simulink model "mb_kol_model"  (R2026b)
settings: Solver=ode4  StopTime=T  FixedStep=dt
values from neighbouring files (symbols this model uses):
  M = mb_param(S)    [dogrula_mb.m]    (also in mb_animasyon.m = mb_param(S);  S.mgl = 0; mb_kareler.m; olcum_oku.m = squeeze(m.Data);  if size(M,2) ~= 6, M = M'; end)
  m = [thm; olc(x(1), S.qM); v; u]    [blok_ayrik.m]    (also in dogrula_b2.m = min(numel(t_s), numel(o.t)); dogrula_b2_dt.m = min(numel(t_s), numel(o.t)); dogrula_elk.m = min(numel(t_s), numel(o.t)); mb_animasyon.m = mean(th(son)))
  S = sim_param(q, D(k).ac, kp)    [deney_4a.m]    (also in dogrula_2.m = sim_param(q, h.ac, ref.kp); dogrula_3.m = sim_param(q, h.ac, kp); dogrula_b2.m = sim_param(q, ac, kp); dogrula_b2_dt.m = sim_param(q, ac, kp))
  s = any(C >= 3 & A > 0.5, 3)    [analiz_5b.m]    (also in blok_ayrik.m = sin(2*pi*S.dny_f0*tau); deney_4a.m = fr > 0.5 & fr < 0.5/dt; km_kestir.m = find(t >= tbas, 1); olcum_4b.m = K.t > 0.1)
  Ts = t(2) - t(1)    [km_kestir.m]    (also in tani_Fs.m; tani_JM.m; tani_JM_kol.m; tani_Ks.m)
  X = squeeze(xs.Data);  if size(X,2) ~= 4, X = X'; end    [deney_4a.m]    (also in dogrula_2.m = squeeze(xs.Data); dogrula_3.m = squeeze(xs.Data); dogrula_5a.m = squeeze(xs.Data); dogrula_b2.m)
  Y = abs(fft(y .* (0.5 - 0.5*cos(2*pi*(0:n-1)'/(n-1)))))    [deney_4a.m]    (also in mb_kareler.m = reshape(P(2,:), size(x)) + c(2))
  Z = reshape(P(3,:), size(x)) + c(3)    [mb_kareler.m]
libraries: sm_lib x15, fl_lib x8, nesl_utility x7
settings Model: Creator=safak  LastModifiedBy=safak
settings DataIOCC: Decimation=dec  SaveTime=off  SignalLogging=off
settings DebuggingCC: AlgebraicLoopMsg=none
settings SimscapeCC: SimscapeLogType=all  SimscapeNominalValues="[{\"value\":\"1\",\"unit\":\"A\"},{\"value\":\"1\",\"unit\":\"bar\"},{\"value\":\"1\",\"unit\":\"cm^2\"},{\"value\":\"1\",\"unit\":\"cm^3/s\"},{\"value\":\"1\",\"unit\":\"kJ/kg\"},{\"value\":\"1\",\"unit\":\"kW\"},{\"value\":\"1\",\"unit\":\"l\"},{\"value\":\"1\",\"unit\":\"N\"},{\"value\":\"1\",\"unit\":\"N*m\"},{\"value\":\"1\",\"unit\":\"V\"},{\"value\":\"0.001\",\"unit\":\"Wb\"}]"  SimscapeUseEnergyAccounting=off

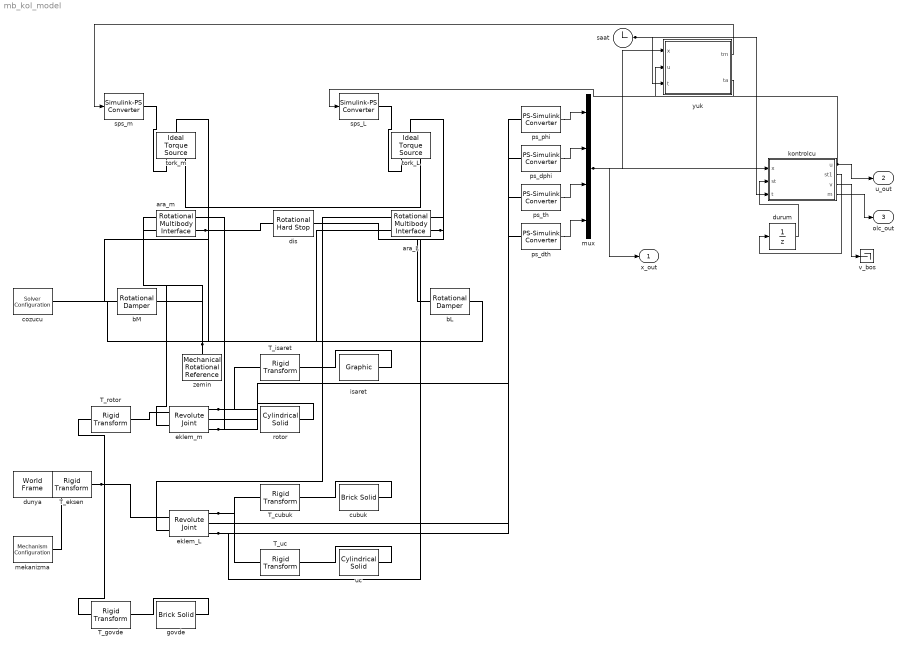
== system mb_kol_model ==
  T_cubuk : sm_lib/Frames and Transforms/Rigid Transform  RotationMethod=None  FollAlignAxisA=+X  BaseAlignAxisA=+Y  FollAlignAxisB=+Y  BaseAlignAxisB=+Z  RotationStandardAxis=+Z  RotationAngle=0  RotationAngleUnits=deg  RotationArbitraryAxis=[0 0 1]  RotationSequenceAxes=FollowerAxes  RotationSequence=XYX  RotationSequenceAngles=[0 0 0]  RotationSequenceAnglesUnits=deg  RotationMatrix=[1 0 0;0 1 0;0 0 1]  Quaternion=[1 0 0 0]  TranslationMethod=Cartesian  TranslationCartesianOffset=[0 -M.L/2 0]  TranslationCartesianOffsetUnits=m  TranslationStandardAxis=+Z  TranslationStandardOffset=0  TranslationStandardOffsetUnits=m  TranslationROffset=0  TranslationROffsetUnits=m  TranslationThetaOffset=0  TranslationThetaOffsetUnits=deg  TranslationZOffset=0  TranslationZOffsetUnits=m
  T_eksen : sm_lib/Frames and Transforms/Rigid Transform  RotationMethod=RotationMatrix  FollAlignAxisA=+X  BaseAlignAxisA=+Y  FollAlignAxisB=+Y  BaseAlignAxisB=+Z  RotationStandardAxis=+Z  RotationAngle=0  RotationAngleUnits=deg  RotationArbitraryAxis=[0 0 1]  RotationSequenceAxes=FollowerAxes  RotationSequence=XYX  RotationSequenceAngles=[0 0 0]  RotationSequenceAnglesUnits=deg  RotationMatrix=[1 0 0; 0 0 -1; 0 1 0]  Quaternion=[1 0 0 0]  TranslationMethod=None  TranslationCartesianOffset=[0 0 0]  TranslationCartesianOffsetUnits=m  TranslationStandardAxis=+Z  TranslationStandardOffset=0  TranslationStandardOffsetUnits=m  TranslationROffset=0  TranslationROffsetUnits=m  TranslationThetaOffset=0  TranslationThetaOffsetUnits=deg  TranslationZOffset=0  TranslationZOffsetUnits=m
  T_govde : sm_lib/Frames and Transforms/Rigid Transform  RotationMethod=None  FollAlignAxisA=+X  BaseAlignAxisA=+Y  FollAlignAxisB=+Y  BaseAlignAxisB=+Z  RotationStandardAxis=+Z  RotationAngle=0  RotationAngleUnits=deg  RotationArbitraryAxis=[0 0 1]  RotationSequenceAxes=FollowerAxes  RotationSequence=XYX  RotationSequenceAngles=[0 0 0]  RotationSequenceAnglesUnits=deg  RotationMatrix=[1 0 0;0 1 0;0 0 1]  Quaternion=[1 0 0 0]  TranslationMethod=Cartesian  TranslationCartesianOffset=[0 0 M.zrot-0.035]  TranslationCartesianOffsetUnits=m  TranslationStandardAxis=+Z  TranslationStandardOffset=0  TranslationStandardOffsetUnits=m  TranslationROffset=0  TranslationROffsetUnits=m  TranslationThetaOffset=0  TranslationThetaOffsetUnits=deg  TranslationZOffset=0  TranslationZOffsetUnits=m
  T_isaret : sm_lib/Frames and Transforms/Rigid Transform  RotationMethod=None  FollAlignAxisA=+X  BaseAlignAxisA=+Y  FollAlignAxisB=+Y  BaseAlignAxisB=+Z  RotationStandardAxis=+Z  RotationAngle=0  RotationAngleUnits=deg  RotationArbitraryAxis=[0 0 1]  RotationSequenceAxes=FollowerAxes  RotationSequence=XYX  RotationSequenceAngles=[0 0 0]  RotationSequenceAnglesUnits=deg  RotationMatrix=[1 0 0;0 1 0;0 0 1]  Quaternion=[1 0 0 0]  TranslationMethod=Cartesian  TranslationCartesianOffset=[0 0.8*M.rrot M.hrot/2]  TranslationCartesianOffsetUnits=m  TranslationStandardAxis=+Z  TranslationStandardOffset=0  TranslationStandardOffsetUnits=m  TranslationROffset=0  TranslationROffsetUnits=m  TranslationThetaOffset=0  TranslationThetaOffsetUnits=deg  TranslationZOffset=0  TranslationZOffsetUnits=m
  T_rotor : sm_lib/Frames and Transforms/Rigid Transform  RotationMethod=None  FollAlignAxisA=+X  BaseAlignAxisA=+Y  FollAlignAxisB=+Y  BaseAlignAxisB=+Z  RotationStandardAxis=+Z  RotationAngle=0  RotationAngleUnits=deg  RotationArbitraryAxis=[0 0 1]  RotationSequenceAxes=FollowerAxes  RotationSequence=XYX  RotationSequenceAngles=[0 0 0]  RotationSequenceAnglesUnits=deg  RotationMatrix=[1 0 0;0 1 0;0 0 1]  Quaternion=[1 0 0 0]  TranslationMethod=Cartesian  TranslationCartesianOffset=[0 0 M.zrot]  TranslationCartesianOffsetUnits=m  TranslationStandardAxis=+Z  TranslationStandardOffset=0  TranslationStandardOffsetUnits=m  TranslationROffset=0  TranslationROffsetUnits=m  TranslationThetaOffset=0  TranslationThetaOffsetUnits=deg  TranslationZOffset=0  TranslationZOffsetUnits=m
  T_uc : sm_lib/Frames and Transforms/Rigid Transform  RotationMethod=None  FollAlignAxisA=+X  BaseAlignAxisA=+Y  FollAlignAxisB=+Y  BaseAlignAxisB=+Z  RotationStandardAxis=+Z  RotationAngle=0  RotationAngleUnits=deg  RotationArbitraryAxis=[0 0 1]  RotationSequenceAxes=FollowerAxes  RotationSequence=XYX  RotationSequenceAngles=[0 0 0]  RotationSequenceAnglesUnits=deg  RotationMatrix=[1 0 0;0 1 0;0 0 1]  Quaternion=[1 0 0 0]  TranslationMethod=Cartesian  TranslationCartesianOffset=[0 -M.d 0]  TranslationCartesianOffsetUnits=m  TranslationStandardAxis=+Z  TranslationStandardOffset=0  TranslationStandardOffsetUnits=m  TranslationROffset=0  TranslationROffsetUnits=m  TranslationThetaOffset=0  TranslationThetaOffsetUnits=deg  TranslationZOffset=0  TranslationZOffsetUnits=m
  ara_L : fl_lib/Mechanical/Multibody Interfaces/Rotational Multibody Interface
  ara_m : fl_lib/Mechanical/Multibody Interfaces/Rotational Multibody Interface
  bL : fl_lib/Mechanical/Rotational Elements/Rotational Damper  D=S.bL N*m*s/rad  w_specify=off  w_priority=None  w=0 rad/s  w_nominal_specify=off  w_nominal_value=1  w_nominal_unit=rad/s  t_specify=off  t_priority=None  t=0 N*m  t_nominal_specify=off  t_nominal_value=1  t_nominal_unit=N*m
  bM : fl_lib/Mechanical/Rotational Elements/Rotational Damper  D=S.bM N*m*s/rad  w_specify=off  w_priority=None  w=0 rad/s  w_nominal_specify=off  w_nominal_value=1  w_nominal_unit=rad/s  t_specify=off  t_priority=None  t=0 N*m  t_nominal_specify=off  t_nominal_value=1  t_nominal_unit=N*m
  cozucu : nesl_utility/Solver Configuration  PhysicalDomain=network_engine_domain  SubClassName=solver  LeftPortType=input  RightPortType=generic  Tones=[]  Harmonics=[]  SimulateNoise=off  Profile=off  UseLocalSampling=off  EnableSwitchedLinearOptims=on  FrequencyDomain=off  UseCCode=off  RelTol=0.001  AbsTol=0.001  MinStep=1e-09  ToWorkspace=off  RevertToSquareIcSolve=off  NumHomotopyIterations=100  PhasorMode=off  PhasorModeNumHarmonics=1  ConsistencySolver=NEWTON_XTOL_AFTER_FTOL  CanonicalOrdering=CANONICAL  OptimizeIntermediates=OPTIMIZED  MulticoreSolverChoice=BACKWARD_EULER  IndexReductionMethod=DerivativeReplacement  DoDC=off  ResidualTolerance=1e-09  ConsistencyTolSource=GLOBAL  ConsistencyAbsTol=0.001  ConsistencyRelTol=0.001  ConsistencyTolFactor=0.001  UseLocalSolver=on  LocalSolverChoice=NE_BACKWARD_EULER_ADVANCER  ResolveIndetEquations=on  FunctionEvalNumThread=1  LocalSolverSampleTime=dt  DoFixedCost=off  MaxNonlinIter=3  MaxModeIter=2  ComputeImpulses=off  ImpulseIterations=2  LinearAlgebra=auto  LinearAlgebraNumThread=0  EquationFormulation=NE_TIME_EF  DelaysMemoryBudget=1024  AutomaticFiltering=on  FilteringTimeConstant=0.001  PartitionStorageMethod=AS_NEEDED  PartitionMemoryBudget=1024  PartitionMethod=BALANCED  MultibodyUseLocalSolver=off  MultibodyLocalSolverChoice=ODE1  MultibodyLocalSolverSampleTime=0.001
  cubuk : sm_lib/Body Elements/Brick Solid  BrickDimensions=[M.w M.L M.t]  BrickDimensionsUnits=m  ExportEntireGeometry=off  InertiaType=Custom  BasedOnType=Density  Density=1000  DensityUnits=kg/m^3  Mass=M.mr  MassUnits=kg  CenterOfMass=[0 0 0]  CenterOfMassUnits=m  MomentsOfInertia=M.Ir  MomentsOfInertiaUnits=kg*m^2  ProductsOfInertia=[0 0 0]  ProductsOfInertiaUnits=kg*m^2  GraphicType=FromGeometry  MarkerShape=Sphere  MarkerSize=10  GraphicVisPropType=SimpleVisualProperties  GraphicDiffuseColor=[0.75 0.78 0.82]  GraphicOpacity=1  GraphicSpecularColor=[0.5 0.5 0.5 1.0]  GraphicAmbientColor=[0.15 0.15 0.15 1.0]  GraphicEmissiveColor=[0.0 0.0 0.0 1.0]  GraphicShininess=75  DoExposeReferenceFrame=on  SerializedFrames=<Frames/>
  dis : fl_lib/Mechanical/Rotational Elements/Rotational Hard Stop  upper_bnd=S.r - (S.x0(1) - S.x0(3)) rad  lower_bnd=-S.r - (S.x0(1) - S.x0(3)) rad  model=simscape.enum.hardstop.smooth  stiff_up=S.Ks N*m/rad  stiff_low=S.Ks N*m/rad  D_up=S.cs N*m*s/rad  D_low=S.cs N*m*s/rad  transition=gecis rad  coeff_rest=0.7  w_tol=0.1 rad/s  trq_tol=0.001 N*m  w_specify=off  w_priority=None  w=0 rad/s  w_nominal_specify=off  w_nominal_value=1  w_nominal_unit=rad/s  t_specify=off  t_priority=None  t=0 N*m  t_nominal_specify=off  t_nominal_value=1  t_nominal_unit=N*m  phi_specify=off  phi_priority=High  phi=0 rad  phi_nominal_specify=off  phi_nominal_value=1  phi_nominal_unit=rad  M_specify=off  M_priority=None  M=0
  dunya : sm_lib/Frames and Transforms/World Frame
  durum : UnitDelay  InitialCondition=S.st0  SampleTime=Ts
  eklem_L : sm_lib/Joints/Revolute Joint  JointMode=Normal  CompositeWrenchDir=FollowerOnBase  CompositeWrenchFrame=BaseFrame  SenseConstraintForce=off  SenseConstraintTorque=off  SenseTotalForce=off  SenseTotalTorque=off  PositionTargetSpecify=on  PositionTargetPriority=High  PositionTargetValue=S.x0(3)  PositionTargetValueUnits=rad  VelocityTargetSpecify=on  VelocityTargetPriority=High  VelocityTargetValue=S.x0(4)  VelocityTargetValueUnits=rad/s  EquilibriumPosition=0  EquilibriumPositionUnits=deg  SpringStiffness=0  SpringStiffnessUnits=N*m/deg  DampingCoefficient=0  DampingCoefficientUnits=N*m/(deg/s)  LowerLimitSpecify=off  LowerLimitBound=-90  LowerLimitBoundUnits=deg  LowerLimitStiffness=1e4  LowerLimitStiffnessUnits=N*m/deg  LowerLimitDamping=10  LowerLimitDampingUnits=N*m/(deg/s)  LowerLimitTransitionRegionWidth=0.1  LowerLimitTransitionRegionWidthUnits=deg  UpperLimitSpecify=off  UpperLimitBound=90  UpperLimitBoundUnits=deg  UpperLimitStiffness=1e4  UpperLimitStiffnessUnits=N*m/deg  UpperLimitDamping=10  UpperLimitDampingUnits=N*m/(deg/s)  UpperLimitTransitionRegionWidth=0.1  UpperLimitTransitionRegionWidthUnits=deg  TorqueActuationMode=InputTorque  MotionActuationMode=ComputedMotion  SensePosition=on  SenseVelocity=on  SenseAcceleration=off  SenseTorqueForce=off  SenseLowerLimitTorqueForce=off  SenseUpperLimitTorqueForce=off
  eklem_m : sm_lib/Joints/Revolute Joint  JointMode=Normal  CompositeWrenchDir=FollowerOnBase  CompositeWrenchFrame=BaseFrame  SenseConstraintForce=off  SenseConstraintTorque=off  SenseTotalForce=off  SenseTotalTorque=off  PositionTargetSpecify=on  PositionTargetPriority=High  PositionTargetValue=S.x0(1)  PositionTargetValueUnits=rad  VelocityTargetSpecify=on  VelocityTargetPriority=High  VelocityTargetValue=S.x0(2)  VelocityTargetValueUnits=rad/s  EquilibriumPosition=0  EquilibriumPositionUnits=deg  SpringStiffness=0  SpringStiffnessUnits=N*m/deg  DampingCoefficient=0  DampingCoefficientUnits=N*m/(deg/s)  LowerLimitSpecify=off  LowerLimitBound=-90  LowerLimitBoundUnits=deg  LowerLimitStiffness=1e4  LowerLimitStiffnessUnits=N*m/deg  LowerLimitDamping=10  LowerLimitDampingUnits=N*m/(deg/s)  LowerLimitTransitionRegionWidth=0.1  LowerLimitTransitionRegionWidthUnits=deg  UpperLimitSpecify=off  UpperLimitBound=90  UpperLimitBoundUnits=deg  UpperLimitStiffness=1e4  UpperLimitStiffnessUnits=N*m/deg  UpperLimitDamping=10  UpperLimitDampingUnits=N*m/(deg/s)  UpperLimitTransitionRegionWidth=0.1  UpperLimitTransitionRegionWidthUnits=deg  TorqueActuationMode=InputTorque  MotionActuationMode=ComputedMotion  SensePosition=on  SenseVelocity=on  SenseAcceleration=off  SenseTorqueForce=off  SenseLowerLimitTorqueForce=off  SenseUpperLimitTorqueForce=off
  govde : sm_lib/Body Elements/Brick Solid  BrickDimensions=[0.05 0.05 0.05]  BrickDimensionsUnits=m  ExportEntireGeometry=off  InertiaType=Custom  BasedOnType=Density  Density=1000  DensityUnits=kg/m^3  Mass=0.2  MassUnits=kg  CenterOfMass=[0 0 0]  CenterOfMassUnits=m  MomentsOfInertia=[1 1 1]*1e-4  MomentsOfInertiaUnits=kg*m^2  ProductsOfInertia=[0 0 0]  ProductsOfInertiaUnits=kg*m^2  GraphicType=FromGeometry  MarkerShape=Sphere  MarkerSize=10  GraphicVisPropType=SimpleVisualProperties  GraphicDiffuseColor=[0.25 0.25 0.28]  GraphicOpacity=1  GraphicSpecularColor=[0.5 0.5 0.5 1.0]  GraphicAmbientColor=[0.15 0.15 0.15 1.0]  GraphicEmissiveColor=[0.0 0.0 0.0 1.0]  GraphicShininess=75  DoExposeReferenceFrame=on  SerializedFrames=<Frames/>
  isaret : sm_lib/Body Elements/Graphic  GraphicType=Marker  MarkerShape=Sphere  MarkerSize=16  GraphicVisPropType=SimpleVisualProperties  GraphicDiffuseColor=[0.05 0.05 0.05]  GraphicOpacity=1  GraphicSpecularColor=[0.5 0.5 0.5 1.0]  GraphicAmbientColor=[0.15 0.15 0.15 1.0]  GraphicEmissiveColor=[0.0 0.0 0.0 1.0]  GraphicShininess=75
  kontrolcu : MATLAB Function  TreatAsAtomicUnit=on
  mekanizma : sm_lib/Utilities/Mechanism Configuration  UniformGravity=Constant  GravityVector=[0 0 -M.g]  GravityVectorUnits=m/s^2  LinearizationDelta=0.001  JointModeTransitionNonlinearIterations=2
  mux : Mux
  ps_dphi : nesl_utility/PS-Simulink Converter  PhysicalDomain=network_engine_domain  SubClassName=ps_output  LeftPortType=input  RightPortType=output  PseudoPeriodic=off  Frequencies=[]  VectorFormat=inherit  Unit=rad/s  AffineConversion=off
  ps_dth : nesl_utility/PS-Simulink Converter  PhysicalDomain=network_engine_domain  SubClassName=ps_output  LeftPortType=input  RightPortType=output  PseudoPeriodic=off  Frequencies=[]  VectorFormat=inherit  Unit=rad/s  AffineConversion=off
  ps_phi : nesl_utility/PS-Simulink Converter  PhysicalDomain=network_engine_domain  SubClassName=ps_output  LeftPortType=input  RightPortType=output  PseudoPeriodic=off  Frequencies=[]  VectorFormat=inherit  Unit=rad  AffineConversion=off
  ps_th : nesl_utility/PS-Simulink Converter  PhysicalDomain=network_engine_domain  SubClassName=ps_output  LeftPortType=input  RightPortType=output  PseudoPeriodic=off  Frequencies=[]  VectorFormat=inherit  Unit=rad  AffineConversion=off
  rotor : sm_lib/Body Elements/Cylindrical Solid  CylinderRadius=M.rrot  CylinderRadiusUnits=m  CylinderLength=M.hrot  CylinderLengthUnits=m  ExportEntireGeometry=off  InertiaType=Custom  BasedOnType=Density  Density=1000  DensityUnits=kg/m^3  Mass=M.mrot  MassUnits=kg  CenterOfMass=[0 0 0]  CenterOfMassUnits=m  MomentsOfInertia=M.Irot  MomentsOfInertiaUnits=kg*m^2  ProductsOfInertia=[0 0 0]  ProductsOfInertiaUnits=kg*m^2  GraphicType=FromGeometry  MarkerShape=Sphere  MarkerSize=10  GraphicVisPropType=SimpleVisualProperties  GraphicDiffuseColor=[0.8 0.45 0.1]  GraphicOpacity=1  GraphicSpecularColor=[0.5 0.5 0.5 1.0]  GraphicAmbientColor=[0.15 0.15 0.15 1.0]  GraphicEmissiveColor=[0.0 0.0 0.0 1.0]  GraphicShininess=75  DoExposeReferenceFrame=on  SerializedFrames=<Frames/>
  saat : Clock
  sps_L : nesl_utility/Simulink-PS Converter  PhysicalDomain=network_engine_domain  SubClassName=ps_input  LeftPortType=input  RightPortType=output  PseudoPeriodic=off  Frequencies=[]  NoiseDistribution=none  NoiseParameters=[]  Unit=N*m  AffineConversion=off  FilteringAndDerivatives=provide  SimscapeFilterOrder=1  InputFilterTimeConstant=0.001  UdotUserProvided=0
  sps_m : nesl_utility/Simulink-PS Converter  PhysicalDomain=network_engine_domain  SubClassName=ps_input  LeftPortType=input  RightPortType=output  PseudoPeriodic=off  Frequencies=[]  NoiseDistribution=none  NoiseParameters=[]  Unit=N*m  AffineConversion=off  FilteringAndDerivatives=provide  SimscapeFilterOrder=1  InputFilterTimeConstant=0.001  UdotUserProvided=0
  tork_L : fl_lib/Mechanical/Mechanical Sources/Ideal Torque Source
  tork_m : fl_lib/Mechanical/Mechanical Sources/Ideal Torque Source
  uc : sm_lib/Body Elements/Cylindrical Solid  CylinderRadius=M.ru  CylinderRadiusUnits=m  CylinderLength=M.hu  CylinderLengthUnits=m  ExportEntireGeometry=off  InertiaType=Custom  BasedOnType=Density  Density=1000  DensityUnits=kg/m^3  Mass=M.mu  MassUnits=kg  CenterOfMass=[0 0 0]  CenterOfMassUnits=m  MomentsOfInertia=M.Iu  MomentsOfInertiaUnits=kg*m^2  ProductsOfInertia=[0 0 0]  ProductsOfInertiaUnits=kg*m^2  GraphicType=FromGeometry  MarkerShape=Sphere  MarkerSize=10  GraphicVisPropType=SimpleVisualProperties  GraphicDiffuseColor=[0.15 0.35 0.7]  GraphicOpacity=1  GraphicSpecularColor=[0.5 0.5 0.5 1.0]  GraphicAmbientColor=[0.15 0.15 0.15 1.0]  GraphicEmissiveColor=[0.0 0.0 0.0 1.0]  GraphicShininess=75  DoExposeReferenceFrame=on  SerializedFrames=<Frames/>
  v_bos : Terminator
  yuk : MATLAB Function  TreatAsAtomicUnit=on
  zemin : fl_lib/Mechanical/Rotational Elements/Mechanical Rotational Reference
  x_out : Outport
  u_out : Outport  Port=2
  olc_out : Outport  Port=3
  wires:
  ps_phi/1 -> mux/1
  ps_dphi/1 -> mux/2
  ps_th/1 -> mux/3
  ps_dth/1 -> mux/4
  mux/1 -> yuk/1(x), kontrolcu/1(x), x_out/1
  kontrolcu/1(u) -> yuk/2(u), u_out/1
  saat/1 -> yuk/3(t), kontrolcu/3(t)
  yuk/1(tm) -> sps_m/1
  yuk/2(ta) -> sps_L/1
  durum/1 -> kontrolcu/2(st)
  kontrolcu/2(st1) -> durum/1
  kontrolcu/3(v) -> v_bos/1
  kontrolcu/4(m) -> olc_out/1
  connections:
  mekanizma/RConn1 -- dunya/RConn1 -- T_eksen/LConn1
  T_govde/LConn1 -- T_eksen/RConn1 -- T_rotor/LConn1 -- eklem_L/LConn1
  T_govde/RConn1 -- govde/RConn1
  T_rotor/RConn1 -- eklem_m/LConn1
  rotor/RConn1 -- eklem_m/RConn1 -- T_isaret/LConn1
  T_isaret/RConn1 -- isaret/RConn1
  T_cubuk/LConn1 -- eklem_L/RConn1 -- T_uc/LConn1
  T_cubuk/RConn1 -- cubuk/RConn1
  T_uc/RConn1 -- uc/RConn1
  cozucu/RConn1 -- ara_m/LConn2 -- ara_L/LConn2 -- bM/RConn1 -- bL/RConn1 -- tork_m/RConn2 -- zemin/LConn1 -- tork_L/RConn2
  ara_m/LConn1 -- eklem_m/LConn2
  ara_m/RConn1 -- eklem_m/RConn3 -- ps_dphi/LConn1
  ara_L/LConn1 -- eklem_L/LConn2
  ara_L/RConn1 -- eklem_L/RConn3 -- ps_dth/LConn1
  dis/LConn1 -- ara_m/RConn2 -- bM/LConn1 -- tork_m/LConn1
  dis/RConn1 -- bL/LConn1 -- ara_L/RConn2 -- tork_L/LConn1
  sps_m/RConn1 -- tork_m/RConn1
  sps_L/RConn1 -- tork_L/RConn1
  eklem_m/RConn2 -- ps_phi/LConn1
  eklem_L/RConn2 -- ps_th/LConn1

== matlab function mb_kol_model/kontrolcu ==
  settings: updateMethod=DISCRETE  sampleTime=Ts
  data: x input; u output; st input; t input; st1 output; v output; m output; S parameter
function [u, st1, v, m] = ayrik(x, st, t, S)
% m: firmware'in Ts'de kaydedeceği ölçümler [th_L (AS5600, gecikmeli); phi (enkoder); v (kestirim); u]
% v: kontrolcünün kullandığı hız (sürücünün zıt EMK kompanzasyonu için dışarı verilir)
% Sensör + kontrolcü, durumsuz yazım (Simscape modeli için). blok_sensor + blok_kontrolcu ile aynı hesap;
% durumlar persistent yerine dışarıdaki Unit Delay'de tutulur: st = [tampon(21); vhat; yprev; z].
% Böylece Simscape ağının (Hard Stop yüzünden) yapısal cebirsel döngüsünü Simulink çözebilir.
%
% Deney kaynağı (firmware'in üreteceği sinyal, Ts örneklemeli; sim_param'daki S.dny_*):
%   S.dny_yer = 0  yok (kontrolcü olduğu gibi)
%               1  referansa eklenir:      e = ref + d - thm          (kapalı çevrim konum uyarımı)
%               2  tork komutuna eklenir:  u0 = kontrolcü + d          (kapalı çevrim tork enjeksiyonu)
%               3  açık çevrim:            u0 = dny_u0 + d, kontrolcü kapalı, integral donuk
%   d = dny_A * şekil(t - dny_t0), yalnız dny_t0 <= t < dny_t0 + dny_Td:
%     S.dny_sek = 1 dikdörtgen (basamak; kısa Td ile darbe), 2 doğrusal chirp f0 -> f1,
%                 3 logaritmik chirp f0 -> f1, 4 sinüs (sabit f0)
%   Serbest salınım: dny_yer = 3, dny_A = 0, dny_u0 = 0 ve başlangıç sapması (p.adim / p.x0).
%
% Hız kestirimi (S.hiz; fv = Inf ise hepsi yerine gerçek hız):
%   0 fark      (y_k - y_{k-1})/Ts + birinci dereceden alçak geçiren (kesim fv)        [varsayılan]
%   1 periyot   son iki enkoder kenarı arasındaki süre: v = n q / (t_kenar - t_önceki_kenar).
%               Kenar zamanı donanımda GPIO kesmesi + µs sayaçla damgalanır; burada iki örnek arasında
%               gerçek açının doğrusal aradeğerlemesiyle bulunur. Yön değişince v = 0. Kenar gelmezse
%               |v| <= q / (t - t_son_kenar) (yavaşlayınca sıfıra iner). Filtre yok.
%   2 gozlemci  ikinci dereceden izleme gözlemcisi (Euler, Ts): e = y - th_hat,
%               th_hat += Ts (w_hat + 2 wo e), w_hat += Ts wo^2 e, wo = 2 pi fv (kritik sönümlü)
% Ek durumlar st(25:28): periyot [phi_önceki (gerçek), t_son_kenar, yön, v]; gozlemci [th_hat, w_hat, 0, 0].
buf = st(1:21);  vhat = st(22);  yprev = st(23);  z = st(24);  ek = st(25:28);
vi = 3;  qv = S.qL;
if S.motorD > 0, vi = 1;  qv = S.qM; end
% --- sensör ---
thm = olc(x(3), S.qL);
if S.gL > 0
    buf = [buf(2:end); thm];
    thm = buf(21 - S.gL);
end
if S.fv_inf > 0
    v = x(vi + 1);
elseif S.hiz == 1
    [v, ek] = periyot(x(vi), t, ek, qv, S.Ts);
    yprev = olc(x(vi), qv);
elseif S.hiz == 2
    yv = olc(x(vi), qv);
    wo = 2*pi*S.fv;
    e_o = yv - ek(1);
    ek(1) = ek(1) + S.Ts*(ek(2) + 2*wo*e_o);
    ek(2) = ek(2) + S.Ts*wo^2*e_o;
    v = ek(2);
    yprev = yv;
else
    yv = olc(x(vi), qv);
    vhat = vhat + S.aV*((yv - yprev)/S.Ts - vhat);
    yprev = yv;
    v = vhat;
end
% --- deney kaynağı ---
d = 0;
if S.dny_yer > 0, d = kaynak(t, S); end
% --- kontrolcü ---
e = S.ref - thm;
if S.dny_yer == 1, e = e + d; end
if S.ppi > 0
    ev = S.kp*e - v;
    u0 = S.KV*ev + S.KI*z;
    iz = ev;
else
    u0 = S.Kp*e + S.Ki*z - S.Kd*v;
    iz = e;
end
if S.dny_yer == 2, u0 = u0 + d; end
acik = S.dny_yer == 3;
if acik, u0 = S.dny_u0 + d; end
u = min(max(u0, -S.Tmax), S.Tmax);
doy = (u0 > S.Tmax && iz > 0) || (u0 < -S.Tmax && iz < 0);
if ~doy && ~acik, z = z + iz*S.Ts; end
if abs(u) < S.olu, u = 0; end
st1 = [buf; vhat; yprev; z; ek];
m = [thm; olc(x(1), S.qM); v; u];   % firmware kaydı: AS5600 (gecikmeli), enkoder, hız kestirimi, tork komutu
end

function [v, ek] = periyot(phi, t, ek, q, Ts)
% ek = [phi_önceki, t_son_kenar, yön, v]. t_son_kenar < 0: henüz kenar yok.
phip = ek(1);  tl = ek(2);  yon = ek(3);  v = ek(4);
n1 = floor(phi/q);  n0 = floor(phip/q);
if n1 ~= n0
    d = sign(n1 - n0);
    if d > 0, sev = n1*q; else, sev = (n1 + 1)*q; end         % son geçilen kenar
    a = (sev - phip)/(phi - phip);  a = min(max(a, 0), 1);
    te = t - Ts + a*Ts;                                        % kenar zamanı (aradeğerleme)
    if d == yon && tl >= 0 && te > tl
        v = d*abs(n1 - n0)*q/(te - tl);
    else
        v = 0;                                                 % ilk kenar ya da yön değişimi
    end
    tl = te;  yon = d;
elseif tl >= 0 && t > tl
    vs = q/(t - tl);                                           % kenar gelmedikçe hız sınırı düşer
    if abs(v) > vs, v = sign(v)*vs; end
end
ek = [phi; tl; yon; v];
end

function y = olc(x, q)
y = x;
if q > 0, y = q*floor(x/q); end
end

function d = kaynak(t, S)
d = 0;
tau = t - S.dny_t0;
if tau < 0 || tau >= S.dny_Td, return; end
switch S.dny_sek
    case 1
        s = 1;
    case 2      % anlık frekans f0 + (f1 - f0) tau / Td
        s = sin(2*pi*(S.dny_f0*tau + (S.dny_f1 - S.dny_f0)*tau^2/(2*S.dny_Td)));
    case 3      % anlık frekans f0 (f1/f0)^(tau/Td)
        k = log(S.dny_f1/S.dny_f0)/S.dny_Td;
        s = sin(2*pi*S.dny_f0*(exp(k*tau) - 1)/k);
    otherwise
        s = sin(2*pi*S.dny_f0*tau);
end
d = S.dny_A*s;
end

== matlab function mb_kol_model/yuk ==
  data: x input; u input; tm output; t input; ta output; S parameter
function [tm, ta] = yuk(x, u, t, S)
% Simscape modelinde fiziksel ağa verilen torklar (Simulink tarafında hesaplanır):
%   tm: motor eylemsizliğine etkiyen net tork = kontrolcü torku - Stribeck sürtünmesi
%   ta: kola etkiyen dış tork = yerçekimi + yük bozucusu
% Viskoz sürtünmeler (bM, bL) ve dişli teması Simscape bloklarındadır.
dphi = x(2);  th = x(3);
tf = 0;
if S.Fc > 0
    tf = (S.Fc + (S.Fs - S.Fc)*exp(-(dphi/S.vs)^2)) * tanh(dphi/S.veps);
end
tm = u - tf;
bz = 0;
if t >= S.d0 && t < S.dT
    bz = S.dA*sin(2*pi*S.df*(t - S.d0));
end
ta = -S.mgl*sin(th) + bz;
end
